simulink model "LQGI_linear_sim"  (R2026a)
settings: Solver=VariableStepAuto
InitFcn:
  | seaDir=fileparts(get_param(bdroot,'FileName'));if isfile(fullfile(seaDir,'..','collaudo_simulink.m')),addpath(fullfile(seaDir,'..'));else,addpath(fullfile(seaDir,'..','..','File_di_Funzioni_Progetto-Accorpati'));end;collaudo_simulink(bdroot);
undefined symbols (not defined in the file): A, Aplant, B, Bplant, C, Cplant, Dplant, Ki, Kx, L, x0plant
settings Model: Creator=rebec  LastModifiedBy=rebec

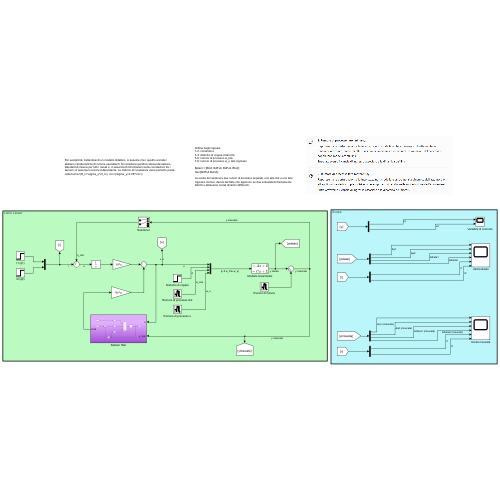
[thumbnail: Simulink's stored preview of the top-level diagram]
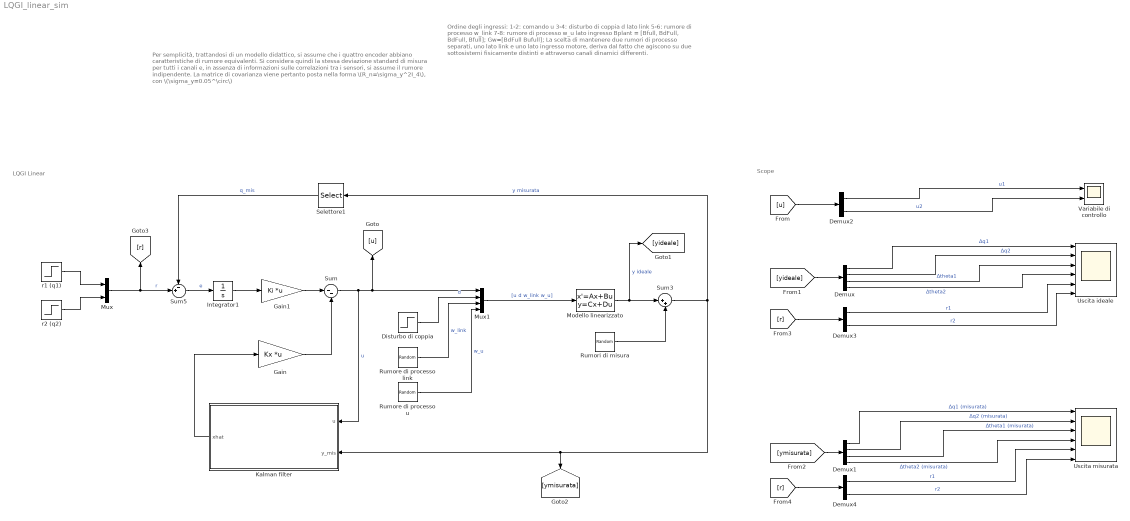
== system LQGI_linear_sim ==
  note: Scope
  note: LQGI Linear
  note: Ordine degli ingressi:
      | 1-2: comando u
      | 3-4: disturbo di coppia d lato link
      | 5-6: rumore di processo w_link
      | 7-8: rumore di processo w_u lato ingresso
      |
      | Bplant = [Bfull, BdFull, BdFull, Bfull];
      | Gw​=[BdFull ​​Bufull​​];
      |
      | La scelta di mantenere due rumori di processo separati, uno lato link e uno lato ingresso motore, deriva dal fatto che agiscono su due sottosistemi fisicamente distinti e attraverso canali dinamici differenti.
  note: Per semplicità, trattandosi di un modello didattico, si assume che i quattro encoder abbiano caratteristiche di rumore equivalenti. Si considera quindi la stessa deviazione standard di misura per tutti i canali e, in assenza di informazioni sulle correlazioni tra i sensori, si assume il rumore indipendente. La matrice di covarianza viene pertanto posta nella forma \(R_n=\sigma_y^2I_4\), con \(\sigma_y=0.05^\circ\)
  Demux : Demux
  Demux1 : Demux
  Demux2 : Demux  Outputs=2
  Demux3 : Demux  Outputs=2
  Demux4 : Demux  Outputs=2
  Disturbo di coppia : Step  Time=[1 1]  InitialValue=[0 0]  FinalValue=[0.5 0]  SampleTime=0
  Gain : Gain  Gain=Kx  Multiplication=Matrix(K*u)
  Gain1 : Gain  Gain=Ki  Multiplication=Matrix(K*u)
  Integrator1 : Integrator
  Kalman filter : Subsystem
  Modello linearizzato : StateSpace  A=Aplant  B=Bplant  C=Cplant  D=Dplant  InitialCondition=x0plant
  Mux : Mux  Inputs=2
  Mux1 : Mux
  Rumore di processo link : RandomNumber  Mean=[0 0]  Variance=[0.01 0.01]  Seed=20260826  SampleTime=0.002
  Rumore di processo u : RandomNumber  Mean=[0 0]  Variance=[0.01 0.01]  Seed=20260826  SampleTime=0.002
  Rumori di misura : RandomNumber  Mean=[0 0 0 0]  Variance=[(0.05*pi/180)^2 (0.05*pi/180)^2 (0.05*pi/180)^2 (0.05*pi/180)^2]  Seed=20260826  SampleTime=0.002
  Selettore1 : Selector  InputPortWidth=4  IndexOptions=Index vector (dialog)  Indices=[1 2]  OutputSizes=1
  Sum : Sum  Inputs=|--
  Sum3 : Sum  Inputs=|++
  Sum5 : Sum  Inputs=-+|
  Uscita ideale : Scope  NumInputPorts=6
      settings: Title=Uscita ideale (LQGI-LIN)  ActiveDisplayYMinimum=-0.32188176451902928  ActiveDisplayYMaximum=0.32726195729465524  YLabel=y (rad)
  Uscita misurata : Scope  NumInputPorts=6
      settings: Title=Uscita misurata (LQGI-LIN)  ActiveDisplayYMinimum=-0.16039480151238891  ActiveDisplayYMaximum=0.22319202869793112  YLabel=y_m_i_s (rad)
  Variabile di controllo : Scope  NumInputPorts=2
      settings: Title=Variabili di controllo (LQGI-LIN)  ActiveDisplayYMinimum=-2.3847906358782209  ActiveDisplayYMaximum=5.4173699379133788  YLabel=u (Nm)  DataLoggingVariableName=ScopeData2
  r1 (q1) : Step  FinalValue=5*pi/180  SampleTime=0
  r2 (q2) : Step  FinalValue=0  SampleTime=0
  wires:
  Gain1/1 -> Sum/1
  Demux/1 -> Uscita ideale/1  "Δq1"
  [r] -> Demux4/1
  Demux/2 -> Uscita ideale/2  "Δq2"
  Mux/1 -> [r], Sum5/2  "r"
  [u] -> Demux2/1
  [yideale] -> Demux/1
  Demux1/3 -> Uscita misurata/3  "Δtheta1 (misurata)"
  Sum3/1 -> Selettore1/1, Kalman filter/2(y_mis), [ymisurata]  "y misurata"
  Demux4/2 -> Uscita misurata/6  "r2"
  Demux4/1 -> Uscita misurata/5  "r1"
  Sum/1 -> Kalman filter/1(u), [u], Mux1/1  "u"
  Demux2/1 -> Variabile di controllo/1  "u1"
  [ymisurata] -> Demux1/1
  Demux/3 -> Uscita ideale/3  "Δtheta1"
  Integrator1/1 -> Gain1/1
  r2 (q2)/1 -> Mux/2
  Gain/1 -> Sum/2
  Demux/4 -> Uscita ideale/4  "Δtheta2"
  Selettore1/1 -> Sum5/1  "q_mis"
  Demux1/2 -> Uscita misurata/2  "Δq2 (misurata)"
  Demux2/2 -> Variabile di controllo/2  "u2"
  Demux3/1 -> Uscita ideale/5  "r1"
  Demux1/1 -> Uscita misurata/1  "Δq1 (misurata)"
  Sum5/1 -> Integrator1/1  "e"
  r1 (q1)/1 -> Mux/1
  Demux3/2 -> Uscita ideale/6  "r2"
  [r] -> Demux3/1
  Demux1/4 -> Uscita misurata/4  "Δtheta2 (misurata)"
  Kalman filter/1(xhat) -> Gain/1
  Modello linearizzato/1 -> [yideale], Sum3/1  "y ideale"
  Mux1/1 -> Modello linearizzato/1  "[u d w_link w_u]"
  Rumori di misura/1 -> Sum3/2
  Disturbo di coppia/1 -> Mux1/2  "d"
  Rumore di processo link/1 -> Mux1/3  "w_link"
  Rumore di processo u/1 -> Mux1/4  "w_u"

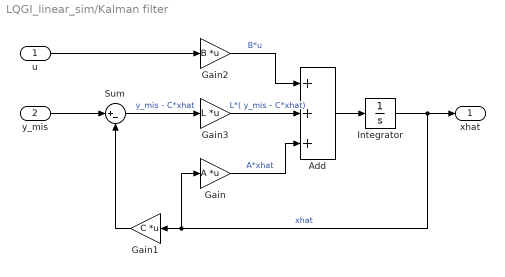
== system LQGI_linear_sim/Kalman filter ==
  u : Inport
  y_mis : Inport  Port=2
  Add : Sum  Inputs=+++
  Gain : Gain  Gain=A  Multiplication=Matrix(K*u)
  Gain1 : Gain  Gain=C  Multiplication=Matrix(K*u)
  Gain2 : Gain  Gain=B  Multiplication=Matrix(K*u)
  Gain3 : Gain  Gain=L  Multiplication=Matrix(K*u)
  Integrator : Integrator
  Sum : Sum  Inputs=|+-
  xhat : Outport
  wires:
  u/1 -> Gain2/1
  y_mis/1 -> Sum/1
  Gain1/1 -> Sum/2
  Sum/1 -> Gain3/1  "y_mis - C*xhat"
  Gain3/1 -> Add/2  "L*( y_mis - C*xhat)"
  Gain2/1 -> Add/1  "B*u"
  Gain/1 -> Add/3  "A*xhat"
  Add/1 -> Integrator/1
  Integrator/1 -> Gain/1, Gain1/1, xhat/1  "xhat"
